simulink library "lib_AC_MGES"  (R2026a)
settings: Solver=VariableStepAuto
undefined symbols (not defined in the file): block_buses, block_fref, block_idx, block_toM, buses_lf, c_fd, c_kd1, c_kq1, c_kq2, fref, gen_static_params, Lbiginv, Lppd_pu, Lppq_pu, op_MGES, Ps_lf, Sb, T_meas_safe
(part 2 of 2)

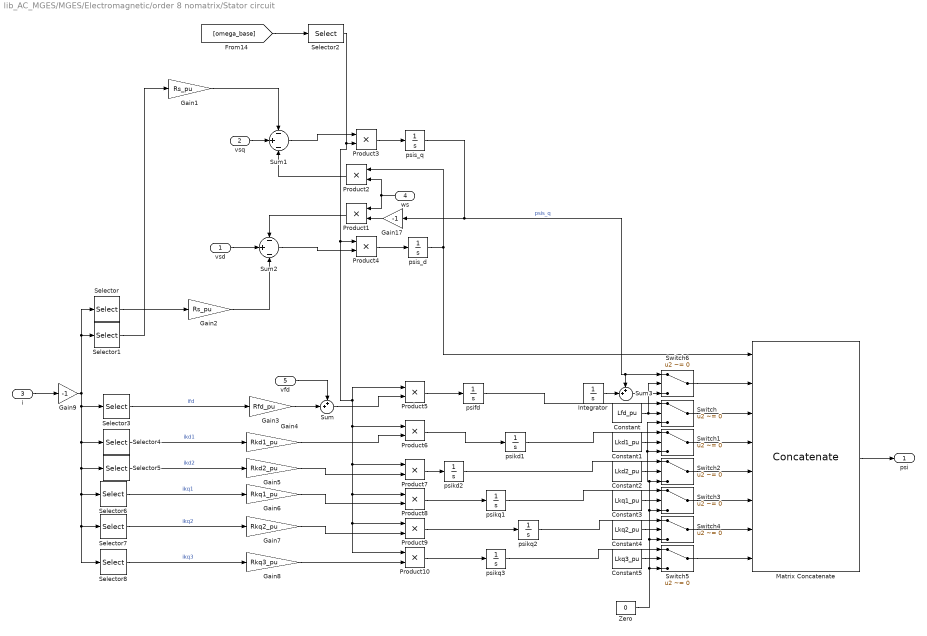
== system lib_AC_MGES/MGES/Electromagnetic/order 8 nomatrix/Stator circuit ==
  vsd : Inport
  vsq : Inport  Port=2
  i : Inport  Port=3
  ws : Inport  Port=4
  vfd : Inport  Port=5
  Constant : Constant  Value=Lfd_pu  VectorParams1D=off
  Constant1 : Constant  Value=Lkd1_pu  VectorParams1D=off
  Constant2 : Constant  Value=Lkd2_pu  VectorParams1D=off
  Constant3 : Constant  Value=Lkq1_pu  VectorParams1D=off
  Constant4 : Constant  Value=Lkq2_pu  VectorParams1D=off
  Constant5 : Constant  Value=Lkq3_pu  VectorParams1D=off
  Gain1 : Gain  Gain=Rs_pu
  Gain17 : Gain  Gain=-1
  Gain2 : Gain  Gain=Rs_pu
  Gain3 : Gain  Gain=Rfd_pu
  Gain4 : Gain  Gain=Rkd1_pu
  Gain5 : Gain  Gain=Rkd2_pu
  Gain6 : Gain  Gain=Rkq1_pu
  Gain7 : Gain  Gain=Rkq2_pu
  Gain8 : Gain  Gain=Rkq3_pu
  Gain9 : Gain  Gain=-1
  Integrator : Integrator  InitialCondition=op_MGES.Electromagnetic_order_8_nomatrix_Stator_circuit_Integr_d80af81f
  Matrix Concatenate : Concatenate  NumInputs=8  Mode=Multidimensional array
  Product{1..10} (10 alike) : Product
  Selector : Selector  NumberOfDimensions=2  InputPortWidth=9  IndexOptions=Index vector (dialog),Select all  Indices=[1],1  OutputSizes=1,1
  Selector1 : Selector  NumberOfDimensions=2  InputPortWidth=9  IndexOptions=Index vector (dialog),Select all  Indices=[2],1  OutputSizes=1,1
  Selector2 : Selector  InputPortWidth=length(fref.ref_units)  IndexOptions=Index vector (dialog)  Indices=block_fref  OutputSizes=1
  Selector3 : Selector  NumberOfDimensions=2  InputPortWidth=9  IndexOptions=Index vector (dialog),Select all  Indices=3,1  OutputSizes=1,1
  Selector4 : Selector  NumberOfDimensions=2  InputPortWidth=9  IndexOptions=Index vector (dialog),Select all  Indices=4,1  OutputSizes=1,1
  Selector5 : Selector  NumberOfDimensions=2  InputPortWidth=9  IndexOptions=Index vector (dialog),Select all  Indices=5,1  OutputSizes=1,1
  Selector6 : Selector  NumberOfDimensions=2  InputPortWidth=9  IndexOptions=Index vector (dialog),Select all  Indices=6,1  OutputSizes=1,1
  Selector7 : Selector  NumberOfDimensions=2  InputPortWidth=9  IndexOptions=Index vector (dialog),Select all  Indices=7,1  OutputSizes=1,1
  Selector8 : Selector  NumberOfDimensions=2  InputPortWidth=9  IndexOptions=Index vector (dialog),Select all  Indices=8,1  OutputSizes=1,1
  Sum : Sum  Inputs=++|
  Sum1 : Sum  Inputs=-|+|-  InputSameDT=on  SaturateOnIntegerOverflow=on  OutDataTypeStr=Inherit: Same as first input
  Sum2 : Sum  Inputs=-|+|-  InputSameDT=on  SaturateOnIntegerOverflow=on  OutDataTypeStr=Inherit: Same as first input
  Sum3 : Sum  Inputs=++|
  Switch{,1..6} (7 alike) : Switch  Criteria=u2 ~= 0  SaturateOnIntegerOverflow=off  InputSameDT=off
  Zero : Constant  Value=0  OutDataTypeStr=Inherit: Inherit via back propagation
  psifd : Integrator  InitialCondition=op_MGES.Electromagnetic_order_8_nomatrix_Stator_circuit_psifd
  psikd1 : Integrator  InitialCondition=op_MGES.Electromagnetic_order_8_nomatrix_Stator_circuit_psikd1
  psikd2 : Integrator  InitialCondition=op_MGES.Electromagnetic_order_8_nomatrix_Stator_circuit_psikd2
  psikq1 : Integrator  InitialCondition=op_MGES.Electromagnetic_order_8_nomatrix_Stator_circuit_psikq1
  psikq2 : Integrator  InitialCondition=op_MGES.Electromagnetic_order_8_nomatrix_Stator_circuit_psikq2
  psikq3 : Integrator  InitialCondition=op_MGES.Electromagnetic_order_8_nomatrix_Stator_circuit_psikq3
  psis_d : Integrator  InitialCondition=op_MGES.Electromagnetic_order_8_nomatrix_Stator_circuit_psis_d
  psis_q : Integrator  InitialCondition=op_MGES.Electromagnetic_order_8_nomatrix_Stator_circuit_psis_q
  psi : Outport  VectorParamsAs1DForOutWhenUnconnected=off
  wires:
  Product3/1 -> psis_q/1
  Sum1/1 -> Product3/1
  Selector3/1 -> Gain3/1  "ifd"
  Selector8/1 -> Gain8/1  "ikq3"
  Selector7/1 -> Gain7/1  "ikq2"
  Selector6/1 -> Gain6/1  "ikq1"
  Selector5/1 -> Gain5/1  "ikd2"
  Selector4/1 -> Gain4/1  "ikd1"
  Gain3/1 -> Sum/2
  vfd/1 -> Sum/1
  Sum/1 -> Product5/2
  Gain4/1 -> Product6/2
  Gain6/1 -> Product8/2
  Gain8/1 -> Product10/2
  Gain7/1 -> Product9/2
  Matrix Concatenate/1 -> psi/1
  i/1 -> Gain9/1
  Product6/1 -> psikd1/1
  Product7/1 -> psikd2/1
  Product8/1 -> psikq1/1
  Product9/1 -> psikq2/1
  Product10/1 -> psikq3/1
  Gain9/1 -> Selector8/1, Selector7/1, Selector6/1, Selector5/1, Selector4/1, Selector3/1, Selector1/1, Selector/1
  vsd/1 -> Sum2/2
  Sum2/1 -> Product4/2
  Product4/1 -> psis_d/1
  ws/1 -> Product1/1, Product2/2
  Gain17/1 -> Product1/2
  psis_q/1 -> Sum3/1, Switch6/1, Gain17/1  "psis_q"
  Product1/1 -> Sum2/1
  Product2/1 -> Sum1/3
  psis_d/1 -> Product2/1, Matrix Concatenate/1
  Selector/1 -> Gain2/1
  Gain2/1 -> Sum2/3
  Selector1/1 -> Gain1/1
  Gain1/1 -> Sum1/1
  vsq/1 -> Sum1/2
  [omega_base] -> Selector2/1
  Selector2/1 -> Product10/1, Product9/1, Product8/1, Product7/1, Product6/1, Product5/1, Product4/1, Product3/2
  Gain5/1 -> Product7/2
  Switch/1 -> Matrix Concatenate/3
  Product5/1 -> psifd/1
  Constant/1 -> Switch6/2, Switch/2
  psifd/1 -> Switch/1
  Zero/1 -> Switch/3, Switch1/3, Switch2/3, Switch3/3, Switch4/3, Switch5/3
  Switch1/1 -> Matrix Concatenate/4
  Switch2/1 -> Matrix Concatenate/5
  Switch3/1 -> Matrix Concatenate/6
  Switch5/1 -> Matrix Concatenate/8
  Switch4/1 -> Matrix Concatenate/7
  psikd1/1 -> Switch1/1
  psikd2/1 -> Switch2/1
  psikq1/1 -> Switch3/1
  psikq2/1 -> Switch4/1
  psikq3/1 -> Switch5/1
  Constant1/1 -> Switch1/2
  Constant2/1 -> Switch2/2
  Constant3/1 -> Switch3/2
  Constant4/1 -> Switch4/2
  Constant5/1 -> Switch5/2
  Switch6/1 -> Matrix Concatenate/2
  Integrator/1 -> Sum3/2
  Sum3/1 -> Switch6/3

== system lib_AC_MGES/MGES/Electromagnetic/order 8 nomatrix/psi->i ==
  psi : Inport
  Constant : Constant  Value=Matrix_flux_to_i
  For Each Subsystem : Subsystem  TreatAsAtomicUnit=on  mask{Matrix_flux_to_i=Matrix_flux_to_i}
  Selector : Selector  NumberOfDimensions=2  InputPortWidth=9  IndexOptions=Index vector (dialog),Select all  Indices=[1],1  OutputSizes=1,1
  Selector1 : Selector  NumberOfDimensions=2  InputPortWidth=9  IndexOptions=Index vector (dialog),Select all  Indices=[2],1  OutputSizes=1,1
  To Workspace : ToWorkspace  VariableName=Matrix_flux_to_i  SaveFormat=Timeseries  SampleTime=-1
  isd : Outport  VectorParamsAs1DForOutWhenUnconnected=off
  i : Outport  Port=2  VectorParamsAs1DForOutWhenUnconnected=off
  isq : Outport  Port=3  VectorParamsAs1DForOutWhenUnconnected=off
  wires:
  Selector/1 -> isd/1
  Selector1/1 -> isq/1
  psi/1 -> For Each Subsystem/1(In1)
  For Each Subsystem/1(Out1) -> Selector1/1, Selector/1, i/1
  Constant/1 -> To Workspace/1

== system lib_AC_MGES/MGES/LeadLag/Active/Impl ==
  In1 : Inport
  AVR_LeadLag : Subsystem  mask{T_2=T_2(T_1~=0), T_1=T_1(T_1~=0)}
      mask help:
      | Transfer function:
      |
      |   1 + sT_2
      | ---------------
      |   1 + sT_1
  Assignment1 : Assignment  DiagnosticForDimensions=Warning  IndexOptions=Index vector (dialog)  Indices=find(T_1~=0)  OutputSizes=1
  Selector10 : Selector  InputPortWidth=length(block_buses)  IndexOptions=Index vector (dialog)  Indices=find(T_1~=0)  OutputSizes=1
  Out1 : Outport
  wires:
  In1/1 -> Selector10/1, Assignment1/1
  Assignment1/1 -> Out1/1
  Selector10/1 -> AVR_LeadLag/1(In1)
  AVR_LeadLag/1(Out1) -> Assignment1/2

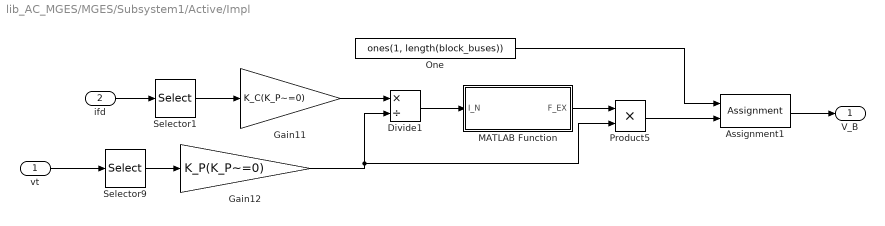
== system lib_AC_MGES/MGES/Subsystem1/Active/Impl ==
  vt : Inport
  ifd : Inport  Port=2
  Assignment1 : Assignment  DiagnosticForDimensions=Warning  IndexOptions=Index vector (dialog)  Indices=find(K_P~=0)  OutputSizes=1
  Divide1 : Product  Inputs=*/
  Gain11 : Gain  Gain=K_C(K_P~=0)
  Gain12 : Gain  Gain=K_P(K_P~=0)
  MATLAB Function : MATLAB Function  TreatAsAtomicUnit=on
  One : Constant  Value=ones(1, length(block_buses))  VectorParams1D=off  OutDataTypeStr=Inherit: Inherit via back propagation
  Product5 : Product
  Selector1 : Selector  InputPortWidth=length(block_buses)  IndexOptions=Index vector (dialog)  Indices=find(K_P~=0)  OutputSizes=1
  Selector9 : Selector  InputPortWidth=length(block_buses)  IndexOptions=Index vector (dialog)  Indices=find(K_P~=0)  OutputSizes=1
  V_B : Outport
  wires:
  Divide1/1 -> MATLAB Function/1(I_N)
  Selector1/1 -> Gain11/1
  ifd/1 -> Selector1/1
  Gain12/1 -> Product5/2, Divide1/2
  MATLAB Function/1(F_EX) -> Product5/1
  Gain11/1 -> Divide1/1
  Selector9/1 -> Gain12/1
  Assignment1/1 -> V_B/1
  vt/1 -> Selector9/1
  One/1 -> Assignment1/1
  Product5/1 -> Assignment1/2

== system lib_AC_MGES/MGES/WOF_d2/Active/Impl ==
  In1 : Inport
  Gain : Gain  Gain=1./max(T_w3, 1e-3)
  I : Integrator  InitialConditionSource=external  InitialCondition=op_MGES.WOF_d2_Active_Impl_I
  Sum : Sum  Inputs=+-|
  Sum4 : Sum  Inputs=|+-
  Out1 : Outport
  wires:
  Sum/1 -> Out1/1
  I/1 -> Sum/2, Sum4/2
  In1/1 -> Sum4/1, Sum/1, I/2
  Sum4/1 -> Gain/1
  Gain/1 -> I/1

== system lib_AC_MGES/MGES/Electromagnetic/order 8 nomatrix/psi->i/For Each Subsystem ==
  In1 : Inport  Partition=on  PartitionDimension=2  PartitionWidth=1  PartitionOffset=0
  For Each : ForEach  DisableCoverage=on  IterateSubsysMaskParameter=on  SubsysMaskParameterIterationDimension=3
  Gain : Gain  Gain=Matrix_flux_to_i  Multiplication=Matrix(K*u)
  Out1 : Outport  ConcatenationDimension=2
  wires:
  In1/1 -> Gain/1
  Gain/1 -> Out1/1

== system lib_AC_MGES/MGES/LeadLag/Active/Impl/AVR_LeadLag ==
  In1 : Inport
  Gain : Gain  Gain=1./T_1
  Gain2 : Gain  Gain=T_2./T_1
  Sum : Sum  Inputs=|+-
  Sum1 : Sum  Inputs=++|
  x_f : Integrator  InitialConditionSource=external  InitialCondition=op_MGES.LeadLag_Active_Impl_AVR_LeadLag_x_f
  Out1 : Outport
  wires:
  In1/1 -> Sum/1, x_f/2
  Sum1/1 -> Out1/1
  Gain2/1 -> Sum1/1
  Sum/1 -> Gain2/1, Gain/1
  Gain/1 -> x_f/1
  x_f/1 -> Sum/2, Sum1/2

== matlab function lib_AC_MGES/MGES/Subsystem1/Active/Impl/MATLAB Function ==
  data: I_N input; F_EX output
function F_EX = fcn_vectorised(I_N)
% This function calculates F_EX based on the value of I_N, element-wise.
% I_N can be a scalar, vector, or matrix.

F_EX = zeros(1, length(I_N)); % Initialize F_EX with zeros, same size as I_N

% Condition 1: I_N <= 0.433
idx1 = (I_N <= 0.433);
F_EX(idx1) = 1 - 0.577 * I_N(idx1);

% Condition 2: 0.433 < I_N <= 0.75
idx2 = (I_N > 0.433) & (I_N <= 0.75);
F_EX(idx2) = sqrt(0.75 - (I_N(idx2)).^2);

% Condition 3: 0.75 < I_N <= 1
idx3 = (I_N > 0.75) & (I_N <= 1);
F_EX(idx3) = 1.732 * (1 - I_N(idx3));

% Condition 4: I_N > 1 (already handled by initialization to zero
% and the fact that previous conditions won't apply)
% No explicit assignment needed here as F_EX is pre-initialized to 0
% for these elements.
end
